simulink model "PV_Unit_day"  (R2025a)
settings: Solver=FixedStepDiscrete  StartTime=0.0  StopTime=24*0.05  FixedStep=Ts  RelTol=1e-3
InitFcn:
  | Ts = 1e-6;
  | t_hour = 0.05;   % simulated seconds per real hour (24 h = 1.2 s)
  | if ~exist('DAY','var'), DAY = 'clear'; end
  | f = fullfile(fileparts(get_param(bdroot,'FileName')), 'pv_daily_profile.mat');
  | if ~isfile(f), f = which('pv_daily_profile.mat'); end
  | S = load(f);   % NASA POWER profile (same folder as the model)
  | t_day = S.t;
  | if strcmp(DAY,'cloudy'), G_day = S.G_cloudy; T_amb_day = S.T_amb_cloudy;
  | else, G_day = S.G_clear; T_amb_day = S.T_amb; end
undefined symbols (not defined in the file or in its folder): G_day
libraries: spsSeriesRLCBranchLib x4, simulink x2, spsVoltageMeasurementLib x2, spsDiodeLib x1, spsCurrentMeasurementLib x1, slpidlib x1, spsPVArrayLib x1, spsIdealSwitchLib x1, spsDCVoltageSourceLib x1, spspowerguiLib x1
settings Model: Creator=JESHNU PRANAV  LastModifiedBy=msssr
settings SolverCC: AutoInsertRateTranBlk=on

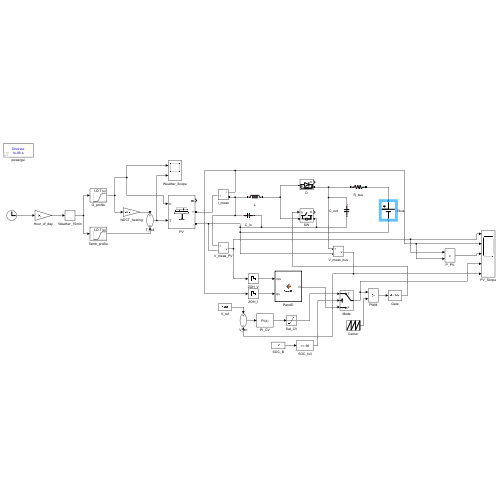
[thumbnail: Simulink's stored preview of the top-level diagram]
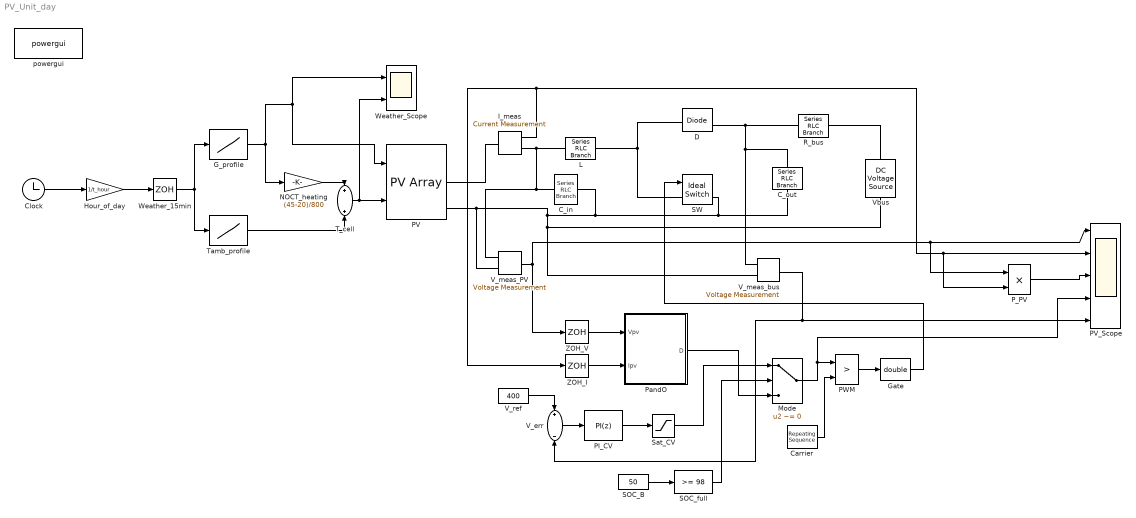
== system PV_Unit_day ==
  C_in : spsSeriesRLCBranchLib/Series RLC Branch  LConnTagsString=__new0  RConnTagsString=__new0  BranchType=C  Resistance=1  Inductance=1e-3  SetiL0=off  InitialCurrent=0  Capacitance=270e-6  Setx0=off  InitialVoltage=0  Measurements=None
  C_out : spsSeriesRLCBranchLib/Series RLC Branch  LConnTagsString=__new0  RConnTagsString=__new0  BranchType=C  Resistance=1  Inductance=1e-3  SetiL0=off  InitialCurrent=0  Capacitance=270e-6  Setx0=off  InitialVoltage=0  Measurements=None
  Carrier : simulink/Sources/Repeating Sequence  rep_seq_t=[0 5e-05]  rep_seq_y=[0 1]
  Clock : Clock
  D : spsDiodeLib/Diode  Ron=0.001  Lon=0  Vf=0.8  IC=0  UseSnubber=0  Rs=500  Cs=250e-9  Measurements=on
  G_profile : Lookup_n-D  NumberOfTableDimensions=1  BreakpointsForDimension1=t_day  Table=G_day  ExtrapMethod=Clip  InternalRulePriority=Speed  RndMeth=Simplest
  Gate : DataTypeConversion  OutDataTypeStr=double  SaturateOnIntegerOverflow=off  RndMeth=Floor
  Hour_of_day : Gain  Gain=1/t_hour
  I_meas : spsCurrentMeasurementLib/Current Measurement  PhasorSimulation=off  OutputType=Complex  PSBequivalent=0
  L : spsSeriesRLCBranchLib/Series RLC Branch  LConnTagsString=__new0  RConnTagsString=__new0  BranchType=L  Resistance=1  Inductance=0.30e-3  SetiL0=off  InitialCurrent=0  Capacitance=1e-6  Setx0=off  InitialVoltage=0  Measurements=None
  Mode : Switch  Criteria=u2 ~= 0  SaturateOnIntegerOverflow=off  InputSameDT=off
  NOCT_heating : Gain  Gain=(45-20)/800
  PI_CV : slpidlib/PID Controller  Controller=PI  Form=Parallel  TimeDomain=Discrete-time  UseExternalTs=off  SampleTime=0.0001  IntegratorMethod=Forward Euler  FilterMethod=Forward Euler  ControllerParametersSource=internal  P=0.001  I=0.05  UseKiTs=off  D=0  UseExternalDerivativeSource=off  N=100  UseFilter=on  TunerSelectOption=Transfer Function Based (PID Tuner App)  InitialConditionSource=internal  InitialConditionForIntegrator=0  InitialConditionForFilter=0  DifferentiatorICPrevScaledInput=0  ExternalReset=none  TrackingMode=off  Kt=1  LimitOutput=off  SatLimitsSource=internal  UpperSaturationLimit=inf  LowerSaturationLimit=-inf  LinearizeAsGain=off  AntiWindupMode=none  Kb=1  LimitIntegrator=off  UpperIntegratorSaturationLimit=inf  LowerIntegratorSaturationLimit=-inf  POutMin=[]  POutMax=[]  IOutMin=[]  IOutMax=[]  DOutMin=[]  DOutMax=[]  NOutMin=[]  NOutMax=[]  SumOutMin=[]  SumOutMax=[]  SaturationOutMin=[]  SaturationOutMax=[]  PParamMin=[]  PParamMax=[]  IParamMin=[]  IParamMax=[]  DParamMin=[]  DParamMax=[]  NParamMin=[]  NParamMax=[]  KbParamMin=[]  KbParamMax=[]  KtParamMin=[]  KtParamMax=[]  KbOutMin=[]  KbOutMax=[]  KtOutMin=[]  KtOutMax=[]  IntegratorOutMin=[]  IntegratorOutMax=[]  FilterOutMin=[]  FilterOutMax=[]  SumI1OutMin=[]  SumI1OutMax=[]  SumI2OutMin=[]  SumI2OutMax=[]  SumI3OutMin=[]  SumI3OutMax=[]  SumI4OutMin=[]  SumI4OutMax=[]  SumDOutMin=[]  SumDOutMax=[]  DifferentiatorOutMin=[]  DifferentiatorOutMax=[]  FilterDiffOutCoefMin=[]  FilterDiffOutCoefMax=[]  ReciprocalOutMin=[]  ReciprocalOutMax=[]  SumDenOutMin=[]  SumDenOutMax=[]  SumNumOutMin=[]  SumNumOutMax=[]  DivideOutMin=[]  DivideOutMax=[]  UdiffTsProdOutMin=[]  UdiffTsProdOutMax=[]  NTsProdOutMin=[]  NTsProdOutMax=[]  UintegralTsProdOutMin=[]  UintegralTsProdOutMax=[]  UngainTsProdOutMin=[]  UngainTsProdOutMax=[]  ClampingZeroOutDataTypeStr=Inherit: Inherit via back propagation  ClampingZeroOutMin=[]  ClampingZeroOutMax=[]  FilterDenConstantOutDataTypeStr=Inherit: Inherit via back propagation  FilterDenConstantOutMin=[]  FilterDenConstantOutMax=[]  PCopyOutDataTypeStr=Inherit: Inherit via back propagation  PCopyOutMin=[]  PCopyOutMax=[]  NCopyOutDataTypeStr=Inherit: Inherit via back propagation  NCopyOutMin=[]  NCopyOutMax=[]  IntegratorContinuousStateAttributes=''  IntegratorStateMustResolveToSignalObject=off  IntegratorRTWStateStorageClass=Auto  FilterContinuousStateAttributes=''  FilterStateMustResolveToSignalObject=off  FilterRTWStateStorageClass=Auto  ParallelPVariant=InternalParameters  IdealPVariant=Disabled  IVariant=InternalParameters  DVariant=Disabled  IntegratorVariant=Discrete  SatVariant=Disabled  AWVariant=Passthrough  PCopyVariant=Disabled  TRVariant=Disabled  FdbkBlocksVariant=Forward  IdealPFdbkVariant=Disabled  SatFdbkVariant=Disabled  DerivativeFilterVariant=Disabled  NVariant=Disabled  NCopyVariant=Disabled_SignalSpec  FilterICVariant=Disabled  IntegratorICVariant=InternalICs  ExternalResetVariant=Disabled  TRSumVariant=Passthrough  SumFdbkVariant=Disabled  SumVariant=Sum_PI  TsampFilterVariant=InternalTs  TsampNgainVariant=Passthrough  TsampIntegralVariant=Disabled_SignalSpec  ExternalSaturationOutDataTypeStr=Inherit: Same as second input  DerivativeSourceVariant=Disabled  PreIntVariant=InternalPreInt
      settings: LibrarySourceBlock=simulink/Discrete/Discrete PID Controller
  PV : spsPVArrayLib/PV Array  Npar=8  Nser=6  PlotType=array @ 1000 W/m2 & specified temperatures  S_vec="[ 1000  500  100 ]"  Temp_C_vec="[ 45 25  ]"  ModuleName=User-defined  PlotWhenSelected=off  Pm=400  Ncell=72  Voc=48  Isc=10.5  Vm=40  Im=10  beta_Voc_pc=-0.36099  alpha_Isc_pc=0.102  beta_Voc=-0.17328  alpha_Isc=0.01071  IL=10.576  I0=3.9433e-10  nI=1.0809  Rsh=821.7644  Rs=0.20021  RobustModel=off  RobustCellTemperature=313.3991  BAL=on  Tc=1e-6  Tfilter=5e-5
  PV_Scope : Scope  NumInputPorts=5
      settings: ActiveDisplayYMinimum=-29.815335077225459  ActiveDisplayYMaximum=268.33801450229595  DataLoggingDecimation=100  DataLoggingVariableName=pvdata
  PWM : RelationalOperator  Operator=>  OutDataTypeStr=boolean  RndMeth=Simplest  InputSameDT=off
  P_PV : Product
  PandO : MATLAB Function  TreatAsAtomicUnit=on
  R_bus : spsSeriesRLCBranchLib/Series RLC Branch  LConnTagsString=__new0  RConnTagsString=__new0  BranchType=R  Resistance=0.1  Inductance=1e-3  SetiL0=off  InitialCurrent=0  Capacitance=1e-6  Setx0=off  InitialVoltage=0  Measurements=None
  SOC_B : Constant  Value=50
  SOC_full : simulink/Logic and Bit Operations/Compare To Constant  relop=>=  const=98  OutDataTypeStr=boolean
  SW : spsIdealSwitchLib/Ideal Switch  Ron=0.001  Lon=0  IC=0  Rs=1e5  Cs=inf  Measurements=on
  Sat_CV : Saturate  UpperLimit=0.85  LowerLimit=0.05
  T_cell : Sum
  Tamb_profile : Lookup_n-D  NumberOfTableDimensions=1  BreakpointsForDimension1=t_day  Table=T_amb_day  ExtrapMethod=Clip  InternalRulePriority=Speed  RndMeth=Simplest
  V_err : Sum  Inputs=+-
  V_meas_PV : spsVoltageMeasurementLib/Voltage Measurement  PhasorSimulation=off  OutputType=Complex  PSBequivalent=0
  V_meas_bus : spsVoltageMeasurementLib/Voltage Measurement  PhasorSimulation=off  OutputType=Complex  PSBequivalent=0
  V_ref : Constant  Value=400
  Vbus : spsDCVoltageSourceLib/DC Voltage Source  Amplitude=400  Measurements=None
  Weather_15min : ZeroOrderHold  SampleTime=t_hour/4
  Weather_Scope : Scope  NumInputPorts=2
      settings: ActiveDisplayYMinimum=-118.6837998765178  ActiveDisplayYMaximum=1068.1541988886604  DataLoggingVariableName=wxdata
  ZOH_I : ZeroOrderHold  SampleTime=0.0001
  ZOH_V : ZeroOrderHold  SampleTime=0.0001
  powergui : spspowerguiLib/powergui  Priority=1  SimulationMode=Discrete  SampleTime=Ts  frequency=60  Iterations=50  frequencyindice=0  Pbase=100e6  ErrMax=1e-4  UnitsV=kV  UnitsW=MW  buscounter=0  FunctionMessages=off  echomessages=off  EnableUseOfTLC=off  CurrentSourceSwitches=off  DisableSnubberDevices=off  DisableRonSwitches=off  DisableVfSwitches=off  DisplayEquations=off  AutomaticDiscreteSolvers=off  SolverType=Tustin/Backward Euler (TBE)  Interpol=off  ExternalGateDelay=off  methode=off  Ts=100  x0status=blocks  SPID=on  SwTol=0  HookPort=off  NonlinearTolerance=1e-4  nMaxIteration=100  ContinueOnMaxIteration=off  RestoreLinks=warning  ResistiveCurrentMeasurement=off  Frange=[0:2:500]  Ylog=off  Xlog=on  ShowGrid=off  save=off  variable=ZData  structure=0  ZoomFFT=off  StartTime=0.0  cycles=1  DisplayStyle=1  fundamental=60  FreqAxis=off  MaxFrequency=1000  frequencyindicesteady=1  RmsSteady=1  display=off
  wires:
  V_meas_PV/1 -> ZOH_V/1, P_PV/1, PV_Scope/1
  I_meas/1 -> P_PV/2, PV_Scope/2, ZOH_I/1
  ZOH_V/1 -> PandO/1(Vpv)
  ZOH_I/1 -> PandO/2(Ipv)
  V_ref/1 -> V_err/1
  V_meas_bus/1 -> V_err/2, PV_Scope/5
  V_err/1 -> PI_CV/1
  PI_CV/1 -> Sat_CV/1
  Sat_CV/1 -> Mode/1
  SOC_B/1 -> SOC_full/1
  SOC_full/1 -> Mode/2
  PandO/1(D) -> Mode/3
  Mode/1 -> PWM/1, PV_Scope/4
  Carrier/1 -> PWM/2
  PWM/1 -> Gate/1
  Gate/1 -> SW/1
  P_PV/1 -> PV_Scope/3
  Clock/1 -> Hour_of_day/1
  Hour_of_day/1 -> Weather_15min/1
  Weather_15min/1 -> G_profile/1, Tamb_profile/1
  G_profile/1 -> PV/1, Weather_Scope/1, NOCT_heating/1
  NOCT_heating/1 -> T_cell/1
  Tamb_profile/1 -> T_cell/2
  T_cell/1 -> Weather_Scope/2, PV/2
  connections:
  PV/RConn1 -- I_meas/LConn1
  C_in/LConn1 -- V_meas_PV/LConn1 -- I_meas/RConn1 -- L/LConn1
  SW/LConn1 -- D/LConn1 -- L/RConn1
  C_out/LConn1 -- V_meas_bus/LConn1 -- D/RConn1 -- R_bus/LConn1
  R_bus/RConn1 -- Vbus/RConn1
  C_in/RConn1 -- PV/RConn2 -- V_meas_PV/LConn2 -- Vbus/LConn1 -- V_meas_bus/LConn2 -- SW/RConn1 -- C_out/RConn1

== matlab function PV_Unit_day/PandO ==
  data: Vpv input; D output; Ipv input
function D = PandO(Vpv, Ipv)
% P&O MPPT with night parking, for a boost converter on a 400 V bus.
% Vpv = (1 - D) * Vbus, so lowering D raises the PV voltage.
persistent Vold Pold Dold
if isempty(Vold), Vold = 0; Pold = 0; Dold = 0.42; end
dD = 0.002;  Pmin = 150;  D_park = 0.42;
P  = Vpv*Ipv;  dV = Vpv - Vold;  dP = P - Pold;
if P < Pmin          % night or very weak light: park near 0.8*Voc
    D = D_park;
elseif dP == 0
    D = Dold;
elseif dP*dV > 0     % left of MPP: raise Vpv by lowering D
    D = Dold - dD;
else                 % right of MPP: lower Vpv by raising D
    D = Dold + dD;
end
% Voltage window: Vpv command 160-256 V (D 0.36-0.60). Covers every MPP
% of the day (~195-245 V) but never asks for more than Voc (~255+ V),
% so P&O cannot drift to open circuit when irradiance rises at sunrise.
D = min(max(D, 0.36), 0.60);
Vold = Vpv; Pold = P; Dold = D;
